simulink model "fcn"  (Simulink 7.1)
settings: Solver=ode45  StartTime=0.0  StopTime=10.0  RelTol=1e-3
settings Model: Creator=W7  LastModifiedBy=W7
settings DataIOCC: ExternalInput=[u]  LoadExternalInput=on

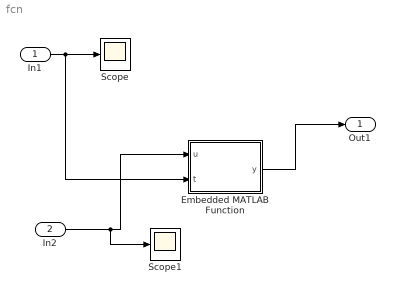
== system fcn ==
  In1 : Inport  OutDataType=sfix(16)  OutScaling=2^0
  In2 : Inport  Port=2  OutDataType=sfix(16)  OutScaling=2^0  Interpolate=off
  Embedded MATLAB Function : Stateflow chart
  Scope : Scope
  Scope1 : Scope
  Out1 : Outport  OutDataType=sfix(16)  OutScaling=2^0
  wires:
  Embedded MATLAB Function/1(y) -> Out1/1
  In2/1 -> Embedded MATLAB Function/1(u), Scope1/1
  In1/1 -> Scope/1, Embedded MATLAB Function/2(t)

== matlab function Embedded MATLAB Function ==
  data: u input double; y output double; t input double
function y = fcn(u,t)
% This block supports the Embedded MATLAB subset.
% See the help menu for details. 

    y= u;
end
